simulink model "kalman_simulink_sim"  (R2026b)
settings: Solver=VariableStepAuto  StopTime=1500
values from neighbouring files (symbols this model uses):
  Ad = sysd.A    [kalman_manuel.m]    (also in kalman_simulink.m)
  Bkal = [Bd Gd]    [kalman_simulink.m]
  C_meas = [1 0 0 0 0 ... (first row only)    [kalman_manuel.m]    (also in kalman_simulink.m)
  D_meas = zeros(2, 2)    [kalman_simulink.m]
  R = [0.245637158512  0; 0  0.335511625509]    [R_from_logs.mat]    (also in estimate_R.m = R_diag; kalman_manuel.m = diag([0.4956^2, 0.5792^2]); kalman_simulink.m = diag([0.4956^2, 0.5792^2]))
  Ts = 1    [R_from_logs.mat]    (also in estimate_R.m; kalman_manuel.m; kalman_simulink.m; model_file.m)
  xhat0 = Tamb * ones(5, 1)    [kalman_simulink.m]
undefined symbols (not defined in the file or in its folder): Discrete, Time
libraries: ctrlSharedLib x1
settings Model: Creator=nael  LastModifiedBy=nael
settings RTWCC: GPUComputeCapability=5.0
settings SimscapeCC: SimscapeUseEnergyAccounting=off

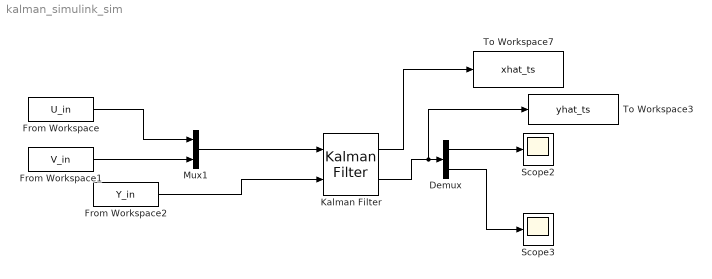
== system kalman_simulink_sim ==
  Demux : Demux  Outputs=2
  From Workspace : FromWorkspace  VariableName=U_in  SampleTime=Ts
  From Workspace1 : FromWorkspace  VariableName=V_in  SampleTime=Ts
  From Workspace2 : FromWorkspace  VariableName=Y_in  SampleTime=Ts
  Kalman Filter : ctrlSharedLib/Kalman Filter  TimeDomain=Discrete-Time  UseCurrentEstimator=on  ModelSource=Individual A, B, C, D matrices  ModelSourceVariable=ss(0.95,1,1,0,1)  A=Ad  B=Bkal  C=C_meas  D=D_meas  NumberOfStates=1  NumberOfInputs=1  NumberOfOutputs=1  Ts=Ts  InitialEstimateSource=Dialog  X0=xhat0  P0=10  UseK=off  UseGH=off  G=1  TimeInvariantG=on  H=0  TimeInvariantH=on  NumberOfProcessNoiseInputs=1  Q=Q  TimeInvariantQ=on  R=R  TimeInvariantR=on  N=0  TimeInvariantN=on  AddInputPort=on  AddEnablePort=off  OutputEstimatedY=on  OutputP=off
  Mux1 : Mux  Inputs=2
  Scope2 : Scope
      settings: ActiveDisplayYMinimum=-1  ActiveDisplayYMaximum=1
  Scope3 : Scope
      settings: ActiveDisplayYMinimum=-1  ActiveDisplayYMaximum=1  DataLoggingVariableName=ScopeData2
  To Workspace3 : ToWorkspace  VariableName=yhat_ts  SaveFormat=Timeseries  SampleTime=Ts
  To Workspace7 : ToWorkspace  VariableName=xhat_ts  SaveFormat=Timeseries  SampleTime=Ts
  wires:
  From Workspace/1 -> Mux1/1
  From Workspace1/1 -> Mux1/2
  Mux1/1 -> Kalman Filter/1
  From Workspace2/1 -> Kalman Filter/2
  Demux/1 -> Scope2/1
  Demux/2 -> Scope3/1
  Kalman Filter/1 -> To Workspace7/1
  Kalman Filter/2 -> To Workspace3/1, Demux/1
